simulink model "PandO"  (R2024a)
settings: Solver=ode15s  StartTime=0.0  StopTime=5  FixedStep=1e-5  MaxStep=0.0001  RelTol=1e-5
values from neighbouring files (symbols this model uses):
  T = T_Array(i)    [CollectData.m]
libraries: spsDiodeLib x4, spsPVArrayLib x3, spsControlledVoltageSourceLib x1, spsCurrentMeasurementLib x1, spsVoltageMeasurementLib x1, spspowerguiLib x1
settings Model: Creator=user  LastModifiedBy=Donald
settings OptimizationCC: DefaultParameterBehavior=Inlined  EnhancedBackFolding=on  PassReuseOutputArgsAs=Individual arguments  ZeroExternalMemoryAtStartup=off  ZeroInternalMemoryAtStartup=off  OptimizeBlockOrder=speed  DifferentSizesBufferReuse=on  OptimizationCustomize=off  EfficientTunableParamExpr=on
settings DebuggingCC: AlgebraicLoopMsg=none  ParameterTunabilityLossMsg=error
settings SFSimCC: MATLABDynamicMemAlloc=off  SimTargetLang=C++
settings RTWCC: Description=Embedded Coder  SystemTargetFile=ert.tlc  TemplateMakefile=ert_default_tmf  Toolchain=Microsoft Visual C++ 2017 v15.0 | CMake/Ninja (64-bit Windows)  BuildConfiguration=Release  TargetLang=C++
settings CodeAppCC: ForceParamTrailComments=on  IgnoreCustomStorageClasses=off  OperatorAnnotations=on  SimulinkDataObjDesc=on  SFDataObjDesc=on  InsertBlockDesc=on
settings ERTTargetCC: TargetLangStandard=C++11 (ISO)  GenerateSampleERTMain=on  CodeInterfacePackaging=C++ class  InlinedParameterPlacement=NonHierarchical  RootIOFormat=Structure reference  ERTCustomFileTemplate=example_file_process.tlc

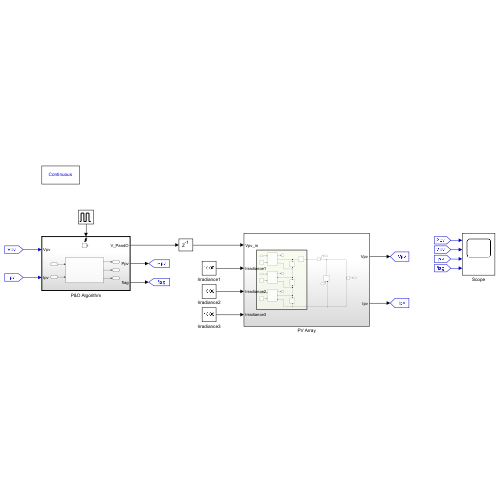
[thumbnail: Simulink's stored preview of the top-level diagram]
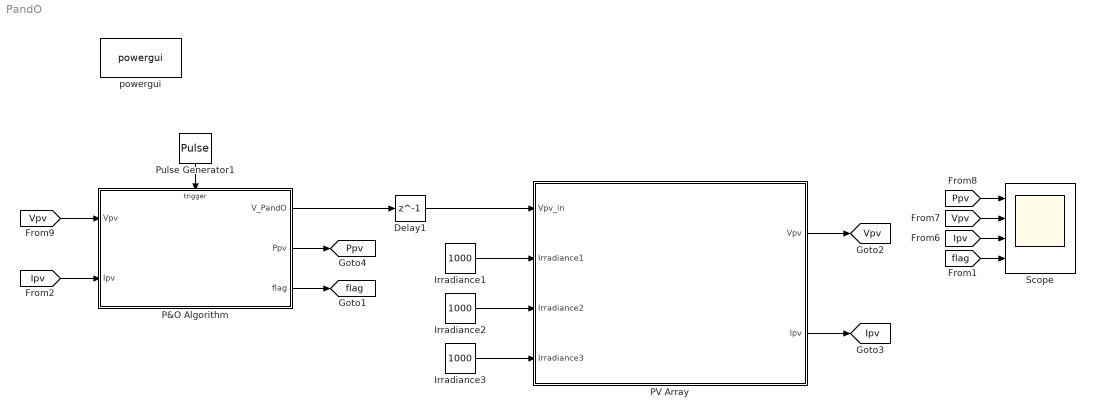
== system PandO ==
  Delay1 : Delay  DelayLength=1
  Irradiance1 : Constant  Value=1000
  Irradiance2 : Constant  Value=1000
  Irradiance3 : Constant  Value=1000
  P&O Algorithm : Subsystem  TreatAsAtomicUnit=on
  PV Array : Subsystem
  Pulse Generator1 : DiscretePulseGenerator  PulseType=Time based  Period=1/1000  PulseWidth=50
  Scope : Scope  NumInputPorts=4
  powergui : spspowerguiLib/powergui  Priority=1  SimulationMode=Continuous  SampleTime=1e-5  frequency=60  Iterations=50  frequencyindice=0  Pbase=100e6  ErrMax=1e-4  UnitsV=kV  UnitsW=MW  buscounter=0  FunctionMessages=on  echomessages=off  EnableUseOfTLC=off  CurrentSourceSwitches=on  DisableSnubberDevices=off  DisableRonSwitches=off  DisableVfSwitches=off  DisplayEquations=off  AutomaticDiscreteSolvers=off  SolverType=Tustin/Backward Euler (TBE)  Interpol=off  ExternalGateDelay=off  methode=off  Ts=100  x0status=blocks  SPID=on  SwTol=0  HookPort=off  NonlinearTolerance=1e-4  nMaxIteration=100  ContinueOnMaxIteration=off  RestoreLinks=warning  ResistiveCurrentMeasurement=off  Frange=[0:2:500]  Ylog=off  Xlog=on  ShowGrid=off  save=off  variable=ZData  structure=0  ZoomFFT=off  StartTime=0.0  cycles=1  DisplayStyle=1  fundamental=60  FreqAxis=off  MaxFrequency=1000  frequencyindicesteady=1  RmsSteady=1  display=off
  tag scope: Ipv=global, Ppv=global, Vpv=global, flag=global
  wires:
  [Ppv] -> Scope/1
  [Ipv] -> Scope/3
  P&O Algorithm/1(V_PandO) -> Delay1/1
  [Ipv] -> P&O Algorithm/2(Ipv)
  Pulse Generator1/1 -> P&O Algorithm/Trigger
  Irradiance1/1 -> PV Array/2(Irradiance1)
  Irradiance2/1 -> PV Array/3(Irradiance2)
  Irradiance3/1 -> PV Array/4(Irradiance3)
  P&O Algorithm/2(Ppv) -> [Ppv]
  P&O Algorithm/3(flag) -> [flag]
  [Vpv] -> Scope/2
  [flag] -> Scope/4
  PV Array/2(Ipv) -> [Ipv]
  PV Array/1(Vpv) -> [Vpv]
  [Vpv] -> P&O Algorithm/1(Vpv)
  Delay1/1 -> PV Array/1(Vpv_in)

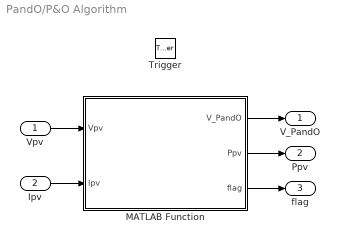
== system PandO/P&O Algorithm ==
  Vpv : Inport
  Ipv : Inport  Port=2
  Trigger : TriggerPort  VariantControl=(inherit)  ShowOutputPort=on
  MATLAB Function : MATLAB Function  TreatAsAtomicUnit=on
  V_PandO : Outport
  Ppv : Outport  Port=2
  flag : Outport  Port=3
  wires:
  Vpv/1 -> MATLAB Function/1(Vpv)
  MATLAB Function/1(V_PandO) -> V_PandO/1
  Ipv/1 -> MATLAB Function/2(Ipv)
  MATLAB Function/2(Ppv) -> Ppv/1
  MATLAB Function/3(flag) -> flag/1

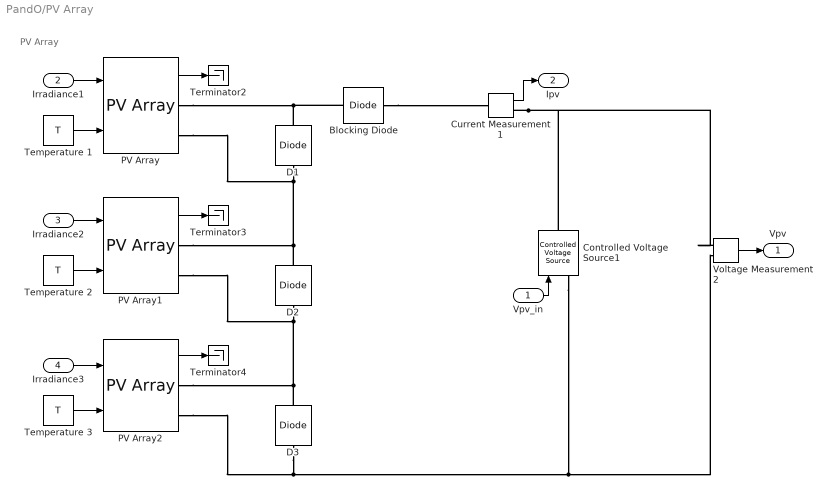
== system PandO/PV Array ==
  note: PV Array
  Vpv_in : Inport
  Irradiance1 : Inport  Port=2
  Irradiance2 : Inport  Port=3
  Irradiance3 : Inport  Port=4
  Blocking Diode : spsDiodeLib/Diode  Ron=0.001  Lon=0  Vf=0.7  IC=0  UseSnubber=off  Rs=1e5*inf  Cs=inf  Measurements=off
  Controlled Voltage Source1 : spsControlledVoltageSourceLib/Controlled Voltage Source  Initialize=on  Source_Type=DC  Amplitude=0  Phase=0  Frequency=0  Measurements=Voltage
  Current Measurement1 : spsCurrentMeasurementLib/Current Measurement  PhasorSimulation=off  OutputType=Complex  PSBequivalent=0
  D1 : spsDiodeLib/Diode  Ron=0.001  Lon=0  Vf=0.7  IC=0  UseSnubber=off  Rs=1e5*inf  Cs=inf  Measurements=off
  D2 : spsDiodeLib/Diode  Ron=0.001  Lon=0  Vf=0.7  IC=0  UseSnubber=off  Rs=1e5*inf  Cs=inf  Measurements=off
  D3 : spsDiodeLib/Diode  Ron=0.001  Lon=0  Vf=0.7  IC=0  UseSnubber=off  Rs=1e5*inf  Cs=inf  Measurements=off
  PV Array : spsPVArrayLib/PV Array  Npar=1  Nser=1  PlotType=array @ 25 deg.C & specified irradiances  S_vec="[ 1000  600  100 ]"  Temp_C_vec="[ 45 25  ]"  ModuleName=User-defined  PlotWhenSelected=off  Pm=83.2824  Ncell=60/3  Voc=37.92*20/60  Isc=8.62  Vm=30.96*20/60  Im=8.07  beta_Voc_pc=-0.36099  alpha_Isc_pc=0.06371  beta_Voc=-0.045629  alpha_Isc=0.0054918  IL=8.6465  I0=3.0335e-10  nI=1.0227  Rsh=76.0432  Rs=0.09434  RobustModel=off  RobustCellTemperature=313.3991  BAL=on  Tc=1e-6  Tfilter=5e-5
  PV Array1 : spsPVArrayLib/PV Array  Npar=1  Nser=1  PlotType=array @ 25 deg.C & specified irradiances  S_vec="[ 1000  600  100 ]"  Temp_C_vec="[ 45 25  ]"  ModuleName=User-defined  PlotWhenSelected=off  Pm=83.2824  Ncell=60/3  Voc=37.92*20/60  Isc=8.62  Vm=30.96*20/60  Im=8.07  beta_Voc_pc=-0.36099  alpha_Isc_pc=0.06371  beta_Voc=-0.045629  alpha_Isc=0.0054918  IL=8.6465  I0=3.0335e-10  nI=1.0227  Rsh=76.0432  Rs=0.09434  RobustModel=off  RobustCellTemperature=313.3991  BAL=on  Tc=1e-6  Tfilter=5e-5
  PV Array2 : spsPVArrayLib/PV Array  Npar=1  Nser=1  PlotType=array @ 25 deg.C & specified irradiances  S_vec="[ 1000  600  100 ]"  Temp_C_vec="[ 45 25  ]"  ModuleName=User-defined  PlotWhenSelected=off  Pm=83.2824  Ncell=60/3  Voc=37.92*20/60  Isc=8.62  Vm=30.96*20/60  Im=8.07  beta_Voc_pc=-0.36099  alpha_Isc_pc=0.06371  beta_Voc=-0.045629  alpha_Isc=0.0054918  IL=8.6465  I0=3.0335e-10  nI=1.0227  Rsh=76.0432  Rs=0.09434  RobustModel=off  RobustCellTemperature=313.3991  BAL=on  Tc=1e-6  Tfilter=5e-5
  Temperature 1 : Constant  Value=T
  Temperature 2 : Constant  Value=T
  Temperature 3 : Constant  Value=T
  Terminator2 : Terminator
  Terminator3 : Terminator
  Terminator4 : Terminator
  Voltage Measurement2 : spsVoltageMeasurementLib/Voltage Measurement  PhasorSimulation=off  OutputType=Complex  PSBequivalent=0
  Vpv : Outport
  Ipv : Outport  Port=2
  wires:
  Irradiance3/1 -> PV Array2/1
  Irradiance2/1 -> PV Array1/1
  Irradiance1/1 -> PV Array/1
  PV Array1/1 -> Terminator3/1
  PV Array/1 -> Terminator2/1
  Temperature 2/1 -> PV Array1/2
  PV Array2/1 -> Terminator4/1
  Temperature 3/1 -> PV Array2/2
  Temperature 1/1 -> PV Array/2
  Vpv_in/1 -> Controlled Voltage Source1/1
  Current Measurement1/1 -> Ipv/1
  Voltage Measurement2/1 -> Vpv/1
  connections:
  D1/RConn1 -- Blocking Diode/LConn1 -- PV Array/RConn1
  D3/RConn1 -- PV Array1/RConn2 -- D2/LConn1 -- PV Array2/RConn1
  PV Array1/RConn1 -- D2/RConn1 -- D1/LConn1 -- PV Array/RConn2
  Blocking Diode/RConn1 -- Current Measurement1/LConn1
  PV Array2/RConn2 -- Voltage Measurement2/LConn2 -- Controlled Voltage Source1/LConn1 -- D3/LConn1
  Current Measurement1/RConn1 -- Controlled Voltage Source1/RConn1 -- Voltage Measurement2/LConn1

== matlab function PandO/P&O Algorithm/MATLAB Function ==
  data: Vpv input; V_PandO output; Ipv input; Ppv output; flag output
function [V_PandO, Ppv, flag] = PandO(Vpv, Ipv)
    % Voltage adjustment step size.
    delta_v = 0.01; 
    
    % Current power.
    Ppv = Vpv * Ipv;
    
    % Persistent variables to retain values between function calls.
    persistent Vold Pold Vcalc stage Voc;

    % Initialize persistent variables on the first function call.
    if isempty(Vcalc)
        stage = 1;
        Voc = 12.64; 
        Vcalc = Voc * 0.4;
        V_PandO = Vcalc;
        Vold = Vpv;
        Pold = Ppv;
        flag = stage;
        return;
    end

    %% Algorithm logic.
    % Enter here when found local max.
    if abs(Ppv - Pold) < 0.001 && (Ppv - Pold) < 0
        V_PandO = Vcalc;
        Vold = Vpv;
        Pold = Ppv;

        % Check if transition to next stage is needed.
        if stage == 1
            Vcalc = Vpv + 0.5;
            stage = stage + 1;
            V_PandO = Vcalc;
        elseif stage == 2
            Vcalc = 0.4 + 1*Voc;
            stage = stage + 1;
            V_PandO = Vcalc;
        elseif stage == 3
            Vcalc = Vpv + 0.5;
            stage = stage + 1;
            V_PandO = Vcalc;
        elseif stage == 4
            Vcalc = 0.4 + 2*Voc;
            stage = stage + 1;
            V_PandO = Vcalc;
        elseif stage == 5
            Vcalc = Vpv + 0.5;
            stage = stage + 1;
            V_PandO = Vcalc;
        elseif stage == 6
            Vcalc = Vcalc + 0;
            stage = stage + 1;
            V_PandO = Vcalc;
        end

    % P&O algorithm.
    else
        % Adjust voltage based on P&O logic.
        if (Ppv - Pold) < 0
            if (Vpv - Vold) < 0
                Vcalc = Vcalc + delta_v;
            else
                Vcalc = Vcalc - delta_v;
            end
        else
            if (Vpv - Vold) < 0
                Vcalc = Vcalc - delta_v;
            else
                Vcalc = Vcalc + delta_v;
            end
        end
        V_PandO = Vcalc;
    end

    % Ensure 'flag' is always defined.
    flag = stage; 

    % Update previous voltage and power for next iteration.
    Vold = Vpv;
    Pold = Ppv;
end
